simulink model "spool_linmod"  (R2026b)
settings: Solver=VariableStepAuto
PostLoadFcn:
  | run(fullfile(fileparts(get_param(bdroot, 'FileName')), 'parameters.m'));
InitFcn:
  | run(fullfile(fileparts(get_param(bdroot, 'FileName')), 'parameters.m'));
values from neighbouring files (symbols this model uses):
  k = 50    [parameters.m]
  n = 2.7    [parameters.m]
  N0 = cases{i,1}    [make_figures.m]
settings Model: Creator=a  LastModifiedBy=a

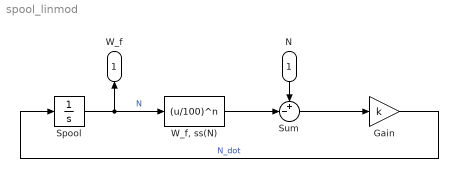
== system spool_linmod ==
  N : Inport
  Gain : Gain  Gain=k
  Spool : Integrator  InitialCondition=N0
  Sum : Sum  Inputs=+-|
  "W_f, ss(N)" : Fcn  Expr=(u/100)^n
  W_f : Outport
  wires:
  Spool/1 -> "W_f, ss(N)"/1, W_f/1  "N"
  "W_f, ss(N)"/1 -> Sum/2
  Sum/1 -> Gain/1
  N/1 -> Sum/1
  Gain/1 -> Spool/1  "N_dot"
